simulink model "PacketizedNetworkSimulinkExample"  (R2025b)
settings: Solver=FixedStepDiscrete  StartTime=0.0  StopTime=200000*Ts  FixedStep=Ts/6  RelTol=1e-3
InitFcn:
  | load networkParams;
  | Ts=1/1e7;
  | ALOHA = 1;
  | CSMA = 0;
  | CA = 1;
values from neighbouring files (symbols this model uses):
  L3payload = [0 0 0 1 0 0 0 0 1 1 1 0 ... (1040 elements, 1040x1)]    [networkParams.mat]
libraries: PacketizedNetworkLib x7, dspsigops x3
Description:
  | This Simulink(R) Model simulates a 3-node wireless network.  Each node in the network has a physical layer and a data link layer of the OSI model.
settings Model: SimulationMode=accelerator  NumberOfSteps=100  Creator=The MathWorks, Inc.  LastModifiedBy=The MathWorks, Inc.
settings SolverCC: AlgebraicLoopSolver=TrustRegion
settings DataIOCC: DSMLogging=off  ReturnWorkspaceOutputs=off
settings OptimizationCC: EfficientMapNaN2IntZero=off
settings DebuggingCC: UnconnectedInputMsg=warning  UnconnectedOutputMsg=warning  UnconnectedLineMsg=warning  ArithmeticOperatorsInVariantConditions=warning
settings HardwareCC: TargetBitPerPointer=64.0  TargetBitPerSizeT=64.0  TargetBitPerPtrDiffT=64.0  TargetLongLongMode=on  TargetIntDivRoundTo=Zero  TargetEndianess=LittleEndian  TargetWordSize=64.0  TargetHWDeviceType=MATLAB Host  ProdEqTarget=off
settings ModelReferenceCC: EnableRefExpFcnMdlSchedulingChecks=on
settings SFSimCC: SimUseLocalCustomCode=off  CustomCodeUndefinedFunction=UseInterfaceOnly
settings RTWCC: RTWUseLocalCustomCode=off  GPUComputeCapability=3.5
settings CodeAppCC: MaxIdLength=128.0  StateflowObjectComments=on
settings GRTTargetCC: TargetLangStandard=C89/C90 (ANSI)  CombineOutputUpdateFcns=off  GRTInterface=on
settings SimscapeCC: SimscapeNormalizeSystem=off

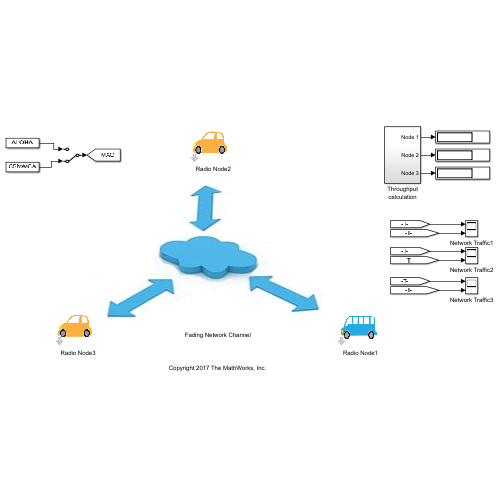
[thumbnail: Simulink's stored preview of the top-level diagram]
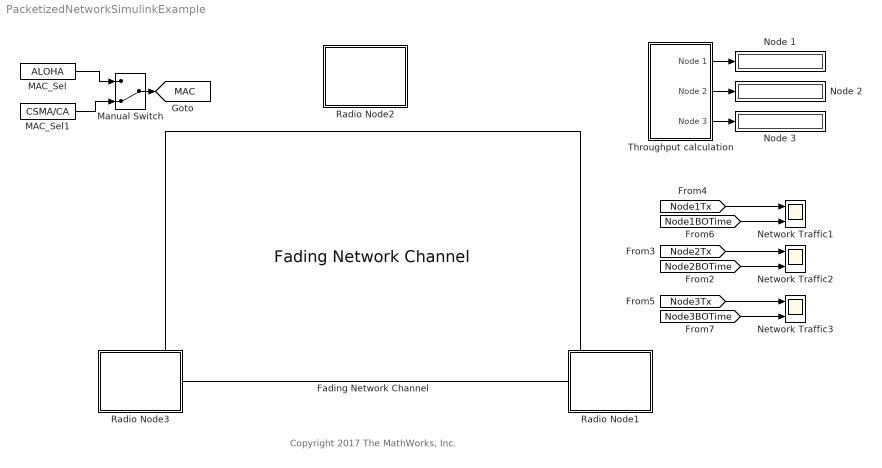
== system PacketizedNetworkSimulinkExample ==
  note: Copyright 2017 The MathWorks, Inc.
  Fading Network Channel : PacketizedNetworkLib/Fading Network Channel  MDSN12=0.00000005/Ts  SNRN12=35  MDSN23=0.00000005/Ts  SNRN23=35  MDSN31=0.00000005/Ts  SNRN31=35
  MAC_Sel : Constant  Value=ALOHA  OutDataTypeStr=boolean  SampleTime=Ts*8
  MAC_Sel1 : Constant  Value=CSMA/CA  OutDataTypeStr=boolean  SampleTime=Ts*8
  Manual Switch : ManualSwitch  CurrentSetting=0
  Network Traffic1 : Scope  NumInputPorts=2
      settings: SampleTime=Ts/(2*3)  Title=Tx 1  ActiveDisplayYMinimum=-0.68347  ActiveDisplayYMaximum=0.68347  DataLoggingVariableName=ScopeData2
  Network Traffic2 : Scope  NumInputPorts=2
      settings: SampleTime=Ts/(2*3)  Title=Tx 2  ActiveDisplayYMinimum=-0.68347  ActiveDisplayYMaximum=0.68347  DataLoggingVariableName=ScopeData2
  Network Traffic3 : Scope  NumInputPorts=2
      settings: SampleTime=Ts/(2*3)  Title=Tx 3  ActiveDisplayYMinimum=-0.68347  ActiveDisplayYMaximum=0.68347
  Node 1 : Display
  Node 2 : Display
  Node 3 : Display
  Radio Node1 : Subsystem  mask{NodeAddre=[0 0 0 0 0 0 0 1], DestAddre=[0 0 0 0 0 0 1 1], AckDestAddre=[0 0 0 0 0 0 1 0], lambda=1e3*8*Ts, pseed=10}
      mask prompts: NodeAddre "Node address:"; DestAddre "Data destination address:"; AckDestAddre "Ack destination address:"; lambda "Arrival rate (arrivals per slot time = 8*Ts):"; pseed "Random seed:"
      mask help:
      | The node address is the ID of the transceiver. The data destination address specifies the recipient of the data packets originating from this transceiver. The Ack destination address specifies the recipient of the acknowledgment packets originating from this transceiver.
      |
      | The lambda parameter regulates the frequency of generated data packets. Higher values specify longer packet interarrival times and therefore less frequent data frame generation.
      settings: NameChangeFcn=|
      | blkName = gcb;
      | set_param([gcb '/From'],'GotoTag',['Node' blkName(end) 'Rx']);
      | set_param([gcb '/Goto'],'GotoTag',['Node' blkName(end) 'Tx']);
      mask DialogControl Container2 Prompt: Parameters
      mask Display:
      | if contains(gcb, 'Node1')
      |   image('Car1.png');
      | else
      |   image('Car2.png');
      | end
  Radio Node2 : Subsystem  mask{NodeAddre=[0 0 0 0 0 0 1 0], DestAddre=[0 0 0 0 0 0 0 1], AckDestAddre=[0 0 0 0 0 0 1 1], lambda=1e3*8*Ts, pseed=13}
      mask prompts: NodeAddre "Node address:"; DestAddre "Data destination address:"; AckDestAddre "Ack destination address:"; lambda "Arrival rate (arrivals per slot time = 8*Ts):"; pseed "Random seed:"
      mask help:
      | The node address is the ID of the transceiver. The data destination address specifies the recipient of the data packets originating from this transceiver. The Ack destination address specifies the recipient of the acknowledgment packets originating from this transceiver.
      |
      | The lambda parameter regulates the frequency of generated data packets. Higher values specify longer packet interarrival times and therefore less frequent data frame generation.
      mask DialogControl Container2 Prompt: Parameters
      mask Display: image('Car2.png');
  Radio Node3 : Subsystem  mask{NodeAddre=[0 0 0 0 0 0 1 1], DestAddre=[0 0 0 0 0 0 1 0], AckDestAddre=[0 0 0 0 0 0 0 1], lambda=1e3*8*Ts, pseed=100}
      mask prompts: NodeAddre "Node address:"; DestAddre "Data destination address:"; AckDestAddre "Ack destination address:"; lambda "Arrival rate (arrivals per slot time = 8*Ts):"; pseed "Random seed:"
      mask help:
      | The node address is the ID of the transceiver. The data destination address specifies the recipient of the data packets originating from this transceiver. The Ack destination address specifies the recipient of the acknowledgment packets originating from this transceiver.
      |
      | The lambda parameter regulates the frequency of generated data packets. Higher values specify longer packet interarrival times and therefore less frequent data frame generation.
      mask Display: image('Car2.png');
  Throughput calculation : Subsystem
  tag scope: MAC=global
  wires:
  MAC_Sel/1 -> Manual Switch/1
  MAC_Sel1/1 -> Manual Switch/2
  Manual Switch/1 -> [MAC]
  [Node1Tx] -> Network Traffic1/1
  [Node1BOTime] -> Network Traffic1/2
  [Node2Tx] -> Network Traffic2/1
  [Node2BOTime] -> Network Traffic2/2
  [Node3Tx] -> Network Traffic3/1
  [Node3BOTime] -> Network Traffic3/2
  Throughput calculation/1(Node 1) -> Node 1/1
  Throughput calculation/2(Node 2) -> Node 2/1
  Throughput calculation/3(Node 3) -> Node 3/1

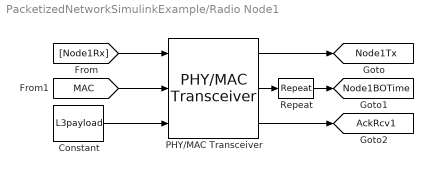
== system PacketizedNetworkSimulinkExample/Radio Node1 ==
  Constant : Constant  Value=L3payload
  PHY/MAC Transceiver : PacketizedNetworkLib/PHY//MAC Transceiver  SystemSampleTime=-1  VariantActivationTime=update diagram  EmptyChoice=off  PassThrough=off  PassThroughVariantControl=(default)  EmptyChoiceVariantControl=(default)  AllowFlexibleInterface=on  Latency=0  AutoFrameSizeCalculation=off
  Repeat : dspsigops/Repeat  FactorSource=Dialog parameter  N=48  Nmax=16  InputProcessing=Columns as channels (frame based)  RateOptions=Allow multirate processing  ic=0  mode=Unused parameter value
  tag scope: AckRcv1=global, Node1BOTime=global, Node1Tx=global
  wires:
  [MAC] -> PHY/MAC Transceiver/2
  PHY/MAC Transceiver/2 -> Repeat/1
  PHY/MAC Transceiver/1 -> [Node1Tx]
  [Node1Rx] -> PHY/MAC Transceiver/1
  Constant/1 -> PHY/MAC Transceiver/3
  Repeat/1 -> [Node1BOTime]
  PHY/MAC Transceiver/3 -> [AckRcv1]

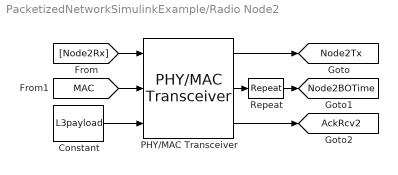
== system PacketizedNetworkSimulinkExample/Radio Node2 ==
  Constant : Constant  Value=L3payload
  PHY/MAC Transceiver : PacketizedNetworkLib/PHY//MAC Transceiver  SystemSampleTime=-1  VariantActivationTime=update diagram  EmptyChoice=off  PassThrough=off  PassThroughVariantControl=(default)  EmptyChoiceVariantControl=(default)  AllowFlexibleInterface=on  Latency=0  AutoFrameSizeCalculation=off
  Repeat : dspsigops/Repeat  FactorSource=Dialog parameter  N=48  Nmax=16  InputProcessing=Columns as channels (frame based)  RateOptions=Allow multirate processing  ic=0  mode=Unused parameter value
  tag scope: AckRcv2=global, Node2BOTime=global, Node2Tx=global
  wires:
  [Node2Rx] -> PHY/MAC Transceiver/1
  PHY/MAC Transceiver/1 -> [Node2Tx]
  [MAC] -> PHY/MAC Transceiver/2
  PHY/MAC Transceiver/2 -> Repeat/1
  Constant/1 -> PHY/MAC Transceiver/3
  Repeat/1 -> [Node2BOTime]
  PHY/MAC Transceiver/3 -> [AckRcv2]

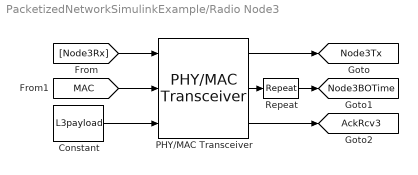
== system PacketizedNetworkSimulinkExample/Radio Node3 ==
  Constant : Constant  Value=L3payload
  PHY/MAC Transceiver : PacketizedNetworkLib/PHY//MAC Transceiver  SystemSampleTime=-1  VariantActivationTime=update diagram  EmptyChoice=off  PassThrough=off  PassThroughVariantControl=(default)  EmptyChoiceVariantControl=(default)  AllowFlexibleInterface=on  Latency=0  AutoFrameSizeCalculation=off
  Repeat : dspsigops/Repeat  FactorSource=Dialog parameter  N=48  Nmax=16  InputProcessing=Columns as channels (frame based)  RateOptions=Allow multirate processing  ic=0  mode=Unused parameter value
  tag scope: AckRcv3=global, Node3BOTime=global, Node3Tx=global
  wires:
  [Node3Rx] -> PHY/MAC Transceiver/1
  PHY/MAC Transceiver/1 -> [Node3Tx]
  [MAC] -> PHY/MAC Transceiver/2
  PHY/MAC Transceiver/2 -> Repeat/1
  Constant/1 -> PHY/MAC Transceiver/3
  Repeat/1 -> [Node3BOTime]
  PHY/MAC Transceiver/3 -> [AckRcv3]

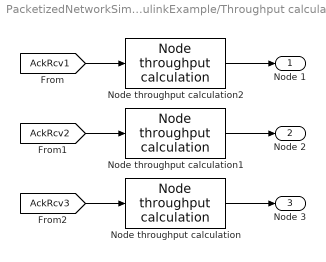
== system PacketizedNetworkSimulinkExample/Throughput calculation ==
  Node throughput calculation : PacketizedNetworkLib/Node throughput calculation  SystemSampleTime=-1  VariantActivationTime=update diagram  EmptyChoice=off  PassThrough=off  PassThroughVariantControl=(default)  EmptyChoiceVariantControl=(default)  AllowFlexibleInterface=on  Latency=0  AutoFrameSizeCalculation=off
  Node throughput calculation1 : PacketizedNetworkLib/Node throughput calculation  SystemSampleTime=-1  VariantActivationTime=update diagram  EmptyChoice=off  PassThrough=off  PassThroughVariantControl=(default)  EmptyChoiceVariantControl=(default)  AllowFlexibleInterface=on  Latency=0  AutoFrameSizeCalculation=off
  Node throughput calculation2 : PacketizedNetworkLib/Node throughput calculation  SystemSampleTime=-1  VariantActivationTime=update diagram  EmptyChoice=off  PassThrough=off  PassThroughVariantControl=(default)  EmptyChoiceVariantControl=(default)  AllowFlexibleInterface=on  Latency=0  AutoFrameSizeCalculation=off
  Node 1 : Outport  VectorParamsAs1DForOutWhenUnconnected=off
  Node 2 : Outport  Port=2  VectorParamsAs1DForOutWhenUnconnected=off
  Node 3 : Outport  Port=3  VectorParamsAs1DForOutWhenUnconnected=off
  wires:
  [AckRcv1] -> Node throughput calculation2/1
  [AckRcv2] -> Node throughput calculation1/1
  Node throughput calculation1/1 -> Node 2/1
  [AckRcv3] -> Node throughput calculation/1
  Node throughput calculation/1 -> Node 3/1
  Node throughput calculation2/1 -> Node 1/1
